simulink model "youBot_Arm_recovery"  (R2024a)
settings: Solver=ode15s  StartTime=0.0  StopTime=20  MaxStep=1e-2  RelTol=1e-3  AbsTol=1e-4
model workspace: external: MATLAB File youBot_DataFile.m (data not in the file)
undefined symbols (not defined in the file): Extr_Data_LinkHoles, Qt, s_curve_home2in, s_curve_in2out, s_curve_out2home, sigbuilder_block, smiData, X, Y, YBT_Par, Z
libraries: sm_lib x193, nesl_utility x130, fl_lib x53, simulink x13, Parts_Lib x10, MyMath_lib x8, Motor_Lib x5, Contact_Forces_Lib x4, ee_lib x2, sdl_lib x2
(part 5 of 8)

== system youBot_Arm_recovery/Arm/Environment/Load/Box ==
  Box : sm_lib/Body Elements/Brick Solid  BrickDimensions=[1 1 1]*YBT_Par.Cube.d  BrickDimensionsUnits=m  ExportEntireGeometry=off  InertiaType=CalculateFromGeometry  BasedOnType=Density  Density=1000  DensityUnits=kg/m^3  Mass=1  MassUnits=kg  CenterOfMass=[0 0 0]  CenterOfMassUnits=m  MomentsOfInertia=[1 1 1]  MomentsOfInertiaUnits=kg*m^2  ProductsOfInertia=[1 1 1]  ProductsOfInertiaUnits=kg*m^2  GraphicType=FromGeometry  MarkerShape=Sphere  MarkerSize=10  GraphicVisPropType=SimpleVisualProperties  GraphicDiffuseColor=[0.4 0.8 1.0]  GraphicOpacity=1.0  GraphicSpecularColor=[0.5 0.5 0.5 1.0]  GraphicAmbientColor=[0.15 0.15 0.15 1.0]  GraphicEmissiveColor=[0.0 0.0 0.0 1.0]  GraphicShininess=75  DoExposeReferenceFrame=on  SerializedFrames=<Frames/>
  Camera Frames : Subsystem
  Init Box 6-DOF Joint : sm_lib/Joints/6-DOF Joint  JointMode=Normal  CompositeWrenchDir=FollowerOnBase  CompositeWrenchFrame=BaseFrame  SenseConstraintForce=off  SenseConstraintTorque=off  SenseTotalForce=off  SenseTotalTorque=off  PxPositionTargetSpecify=off  PxPositionTargetPriority=High  PxPositionTargetValue=0  PxPositionTargetValueUnits=m  PxVelocityTargetSpecify=off  PxVelocityTargetPriority=High  PxVelocityTargetValue=0  PxVelocityTargetValueUnits=m/s  PxEquilibriumPosition=0  PxEquilibriumPositionUnits=m  PxSpringStiffness=0  PxSpringStiffnessUnits=N/m  PxDampingCoefficient=0  PxDampingCoefficientUnits=N/(m/s)  PxLowerLimitSpecify=off  PxLowerLimitBound=-1  PxLowerLimitBoundUnits=m  PxLowerLimitStiffness=1e6  PxLowerLimitStiffnessUnits=N/m  PxLowerLimitDamping=1e3  PxLowerLimitDampingUnits=N/(m/s)  PxLowerLimitTransitionRegionWidth=1e-4  PxLowerLimitTransitionRegionWidthUnits=m  PxUpperLimitSpecify=off  PxUpperLimitBound=1  PxUpperLimitBoundUnits=m  PxUpperLimitStiffness=1e6  PxUpperLimitStiffnessUnits=N/m  PxUpperLimitDamping=1e3  PxUpperLimitDampingUnits=N/(m/s)  PxUpperLimitTransitionRegionWidth=1e-4  PxUpperLimitTransitionRegionWidthUnits=m  PxTorqueActuationMode=NoTorque  PxMotionActuationMode=ComputedMotion  PxSensePosition=off  PxSenseVelocity=off  PxSenseAcceleration=off  PxSenseTorqueForce=off  PxSenseLowerLimitTorqueForce=off  PxSenseUpperLimitTorqueForce=off  PyPositionTargetSpecify=on  PyPositionTargetPriority=High  PyPositionTargetValue=YBT_Par.Cube.init_y  PyPositionTargetValueUnits=m  PyVelocityTargetSpecify=off  PyVelocityTargetPriority=High  PyVelocityTargetValue=0  PyVelocityTargetValueUnits=m/s  PyEquilibriumPosition=0  PyEquilibriumPositionUnits=m  PySpringStiffness=0  PySpringStiffnessUnits=N/m  PyDampingCoefficient=0  PyDampingCoefficientUnits=N/(m/s)  PyLowerLimitSpecify=off  PyLowerLimitBound=-1  PyLowerLimitBoundUnits=m  PyLowerLimitStiffness=1e6  PyLowerLimitStiffnessUnits=N/m  PyLowerLimitDamping=1e3  PyLowerLimitDampingUnits=N/(m/s)  PyLowerLimitTransitionRegionWidth=1e-4  PyLowerLimitTransitionRegionWidthUnits=m  PyUpperLimitSpecify=off  PyUpperLimitBound=1  PyUpperLimitBoundUnits=m  PyUpperLimitStiffness=1e6  PyUpperLimitStiffnessUnits=N/m  PyUpperLimitDamping=1e3  PyUpperLimitDampingUnits=N/(m/s)  PyUpperLimitTransitionRegionWidth=1e-4  PyUpperLimitTransitionRegionWidthUnits=m  PyTorqueActuationMode=NoTorque  PyMotionActuationMode=ComputedMotion  PySensePosition=off  PySenseVelocity=off  PySenseAcceleration=off  PySenseTorqueForce=off  PySenseLowerLimitTorqueForce=off  PySenseUpperLimitTorqueForce=off  PzPositionTargetSpecify=on  PzPositionTargetPriority=High  PzPositionTargetValue=(YBT_Par.Cube.d)/2+YBT_Par.Cube.init_z  PzPositionTargetValueUnits=m  PzVelocityTargetSpecify=off  PzVelocityTargetPriority=High  PzVelocityTargetValue=0  PzVelocityTargetValueUnits=m/s  PzEquilibriumPosition=0  PzEquilibriumPositionUnits=m  PzSpringStiffness=0  PzSpringStiffnessUnits=N/m  PzDampingCoefficient=0  PzDampingCoefficientUnits=N/(m/s)  PzLowerLimitSpecify=off  PzLowerLimitBound=-1  PzLowerLimitBoundUnits=m  PzLowerLimitStiffness=1e6  PzLowerLimitStiffnessUnits=N/m  PzLowerLimitDamping=1e3  PzLowerLimitDampingUnits=N/(m/s)  PzLowerLimitTransitionRegionWidth=1e-4  PzLowerLimitTransitionRegionWidthUnits=m  PzUpperLimitSpecify=off  PzUpperLimitBound=1  PzUpperLimitBoundUnits=m  PzUpperLimitStiffness=1e6  PzUpperLimitStiffnessUnits=N/m  PzUpperLimitDamping=1e3  PzUpperLimitDampingUnits=N/(m/s)  PzUpperLimitTransitionRegionWidth=1e-4  PzUpperLimitTransitionRegionWidthUnits=m  PzTorqueActuationMode=NoTorque  PzMotionActuationMode=ComputedMotion  PzSensePosition=off  PzSenseVelocity=off  PzSenseAcceleration=off  PzSenseTorqueForce=off  PzSenseLowerLimitTorqueForce=off  PzSenseUpperLimitTorqueForce=off  SphPositionTargetSpecify=on  SphPositionTargetPriority=High  SphPositionTargetRotationMethod=StandardAxis  SphPositionTargetFollAlignAxisA=+X  SphPositionTargetBaseAlignAxisA=+Y  SphPositionTargetFollAlignAxisB=+Y  SphPositionTargetBaseAlignAxisB=+Z  SphPositionTargetRotationStandardAxis=+X  SphPositionTargetRotationAngle=0  SphPositionTargetRotationAngleUnits=deg  SphPositionTargetRotationArbitraryAxis=[0 0 1]  SphPositionTargetRotationSequenceAxes=FollowerAxes  SphPositionTargetRotationSequence=XYX  SphPositionTargetRotationSequenceAngles=[0 0 0]  SphPositionTargetRotationSequenceAnglesUnits=deg  SphPositionTargetRotationMatrix=[1 0 0; 0 1 0; 0 0 1]  SphPositionTargetQuaternion=[1 0 0 0]  SphVelocityTargetSpecify=off  SphVelocityTargetPriority=High  SphVelocityTargetValue=[0 0 0]  SphVelocityTargetValueUnits=deg/s  SphVelocityTargetInFollowerFrame=on  SphEqPosRotationMethod=None  SphEqPosFollAlignAxisA=+X  SphEqPosBaseAlignAxisA=+Y  SphEqPosFollAlignAxisB=+Y  SphEqPosBaseAlignAxisB=+Z  SphEqPosRotationStandardAxis=+Z  SphEqPosRotationAngle=0.0  SphEqPosRotationAngleUnits=deg  SphEqPosRotationArbitraryAxis=[0 0 1]  SphEqPosRotationSequenceAxes=FollowerAxes  SphEqPosRotationSequence=XYX  SphEqPosRotationSequenceAngles=[0 0 0]  SphEqPosRotationSequenceAnglesUnits=deg  SphEqPosRotationMatrix=[1 0 0; 0 1 0; 0 0 1]  SphEqPosQuaternion=[1 0 0 0]  SphSpringStiffness=0  SphSpringStiffnessUnits=N*m/deg  SphDampingCoefficient=0  SphDampingCoefficientUnits=N*m/(deg/s)  SphLowerLimitSpecify=off  SphLowerLimitBound=15  SphLowerLimitBoundUnits=deg  SphLowerLimitStiffness=1e4  SphLowerLimitStiffnessUnits=N*m/deg  SphLowerLimitDamping=10  SphLowerLimitDampingUnits=N*m/(deg/s)  SphLowerLimitTransitionRegionWidth=0.1  SphLowerLimitTransitionRegionWidthUnits=deg  SphUpperLimitSpecify=off  SphUpperLimitBound=45  SphUpperLimitBoundUnits=deg  SphUpperLimitStiffness=1e4  SphUpperLimitStiffnessUnits=N*m/deg  SphUpperLimitDamping=10  SphUpperLimitDampingUnits=N*m/(deg/s)  SphUpperLimitTransitionRegionWidth=0.1  SphUpperLimitTransitionRegionWidthUnits=deg  SphTorqueActuationMode=NoTorque  SphActuateTorqueX=off  SphActuateTorqueY=off  SphActuateTorqueZ=off  SphActuateTorque=off  SphActuationFrame=BaseFrame  SphSensePosition=off  SphSenseVelocityX=off  SphSenseVelocityY=off  SphSenseVelocityZ=off  SphSenseVelocity=off  SphSenseAccelerationX=off  SphSenseAccelerationY=off  SphSenseAccelerationZ=off  SphSenseAcceleration=off  SphSenseLowerLimitTorqueMag=off  SphSenseUpperLimitTorqueMag=off  SphSensingFrame=BaseFrame
  Marks : Subsystem
  Transform Face nx : sm_lib/Frames and Transforms/Rigid Transform  RotationMethod=StandardAxis  FollAlignAxisA=+X  BaseAlignAxisA=+Y  FollAlignAxisB=+Y  BaseAlignAxisB=+Z  RotationStandardAxis=+Y  RotationAngle=-90  RotationAngleUnits=deg  RotationArbitraryAxis=[0 0 1]  RotationSequenceAxes=FollowerAxes  RotationSequence=XYX  RotationSequenceAngles=[0 0 0]  RotationSequenceAnglesUnits=deg  RotationMatrix=[1 0 0; 0 1 0; 0 0 1]  Quaternion=[1 0 0 0]  TranslationMethod=None  TranslationCartesianOffset=[0 0 0]  TranslationCartesianOffsetUnits=m  TranslationStandardAxis=+Z  TranslationStandardOffset=0  TranslationStandardOffsetUnits=m  TranslationROffset=0  TranslationROffsetUnits=m  TranslationThetaOffset=0  TranslationThetaOffsetUnits=deg  TranslationZOffset=0  TranslationZOffsetUnits=m
  Transform Face px : sm_lib/Frames and Transforms/Rigid Transform  RotationMethod=StandardAxis  FollAlignAxisA=+X  BaseAlignAxisA=+Y  FollAlignAxisB=+Y  BaseAlignAxisB=+Z  RotationStandardAxis=+Y  RotationAngle=90  RotationAngleUnits=deg  RotationArbitraryAxis=[0 0 1]  RotationSequenceAxes=FollowerAxes  RotationSequence=XYX  RotationSequenceAngles=[0 0 0]  RotationSequenceAnglesUnits=deg  RotationMatrix=[1 0 0; 0 1 0; 0 0 1]  Quaternion=[1 0 0 0]  TranslationMethod=None  TranslationCartesianOffset=[0 0 0]  TranslationCartesianOffsetUnits=m  TranslationStandardAxis=+Z  TranslationStandardOffset=0  TranslationStandardOffsetUnits=m  TranslationROffset=0  TranslationROffsetUnits=m  TranslationThetaOffset=0  TranslationThetaOffsetUnits=deg  TranslationZOffset=0  TranslationZOffsetUnits=m
  Fa : PMIOPort  Side=Right
  Ctr : PMIOPort  Port=2  Side=Left
  Fb : PMIOPort  Port=3  Side=Right
  W : PMIOPort  Port=4  Side=Left
  connections:
  Init Box 6-DOF Joint/LConn1 -- W/RConn1
  Box/RConn1 -- Transform Face px/LConn1 -- Transform Face nx/LConn1 -- Ctr/RConn1 -- Init Box 6-DOF Joint/RConn1 -- Marks/LConn1 -- Camera Frames/LConn1
  Fb/RConn1 -- Transform Face nx/RConn1
  Fa/RConn1 -- Transform Face px/RConn1

== system youBot_Arm_recovery/Arm/Environment/Load/None ==
  Invisible Mass : sm_lib/Body Elements/Brick Solid  BrickDimensions=[1 1 1]  BrickDimensionsUnits=cm  ExportEntireGeometry=off  InertiaType=CalculateFromGeometry  BasedOnType=Density  Density=1000  DensityUnits=kg/m^3  Mass=1  MassUnits=kg  CenterOfMass=[0 0 0]  CenterOfMassUnits=m  MomentsOfInertia=[1 1 1]  MomentsOfInertiaUnits=kg*m^2  ProductsOfInertia=[1 1 1]  ProductsOfInertiaUnits=kg*m^2  GraphicType=FromGeometry  MarkerShape=Sphere  MarkerSize=10  GraphicVisPropType=SimpleVisualProperties  GraphicDiffuseColor=[0.5 0.5 0.5]  GraphicOpacity=0  GraphicSpecularColor=[0.5 0.5 0.5 1.0]  GraphicAmbientColor=[0.15 0.15 0.15 1.0]  GraphicEmissiveColor=[0.0 0.0 0.0 1.0]  GraphicShininess=75  DoExposeReferenceFrame=on  SerializedFrames=<Frames/>
  Transform Box : sm_lib/Frames and Transforms/Rigid Transform  RotationMethod=None  FollAlignAxisA=+X  BaseAlignAxisA=+Y  FollAlignAxisB=+Y  BaseAlignAxisB=+Z  RotationStandardAxis=+Z  RotationAngle=0.0  RotationAngleUnits=deg  RotationArbitraryAxis=[0 0 1]  RotationSequenceAxes=FollowerAxes  RotationSequence=XYX  RotationSequenceAngles=[0 0 0]  RotationSequenceAnglesUnits=deg  RotationMatrix=[1 0 0; 0 1 0; 0 0 1]  Quaternion=[1 0 0 0]  TranslationMethod=Cartesian  TranslationCartesianOffset=[0 YBT_Par.Cube.init_y YBT_Par.Cube.init_z+YBT_Par.Cube.d/2]  TranslationCartesianOffsetUnits=m  TranslationStandardAxis=+Z  TranslationStandardOffset=0  TranslationStandardOffsetUnits=m  TranslationROffset=0  TranslationROffsetUnits=m  TranslationThetaOffset=0  TranslationThetaOffsetUnits=deg  TranslationZOffset=0  TranslationZOffsetUnits=m
  Fa : PMIOPort  Side=Right
  Ctr : PMIOPort  Port=2  Side=Left
  Fb : PMIOPort  Port=3  Side=Right
  W : PMIOPort  Port=4  Side=Left
  connections:
  Transform Box/RConn1 -- Invisible Mass/RConn1 -- Ctr/RConn1
  Transform Box/LConn1 -- W/RConn1

== system youBot_Arm_recovery/Input/Control/Joint Commands/BeltIn to BeltOut ==
  t : Inport
  Bicep : Lookup_n-D  NumberOfTableDimensions=1  LookupTableObject=''  BreakpointsForDimension1=s_curve_in2out.t  Table=s_curve_in2out.q(2,:)  InterpMethod=Cubic spline  ExtrapMethod=Clip  InternalRulePriority=Speed  RndMeth=Simplest
  Forearm : Lookup_n-D  NumberOfTableDimensions=1  LookupTableObject=''  BreakpointsForDimension1=s_curve_in2out.t  Table=s_curve_in2out.q(3,:)  InterpMethod=Cubic spline  ExtrapMethod=Clip  InternalRulePriority=Speed  RndMeth=Simplest
  Gripper : Lookup_n-D  NumberOfTableDimensions=1  LookupTableObject=''  BreakpointsForDimension1=in2out.t  Table=in2out.q(5,:)  InterpMethod=Cubic spline  ExtrapMethod=Clip  InternalRulePriority=Speed  RndMeth=Simplest
  Mux : Mux  Inputs=5
  Pivot : Lookup_n-D  NumberOfTableDimensions=1  LookupTableObject=''  BreakpointsForDimension1=s_curve_in2out.t  Table=s_curve_in2out.q(1,:)  InterpMethod=Cubic spline  ExtrapMethod=Clip  InternalRulePriority=Speed  RndMeth=Simplest
  Wrist : Lookup_n-D  NumberOfTableDimensions=1  LookupTableObject=''  BreakpointsForDimension1=s_curve_in2out.t  Table=s_curve_in2out.q(4,:)  InterpMethod=Cubic spline  ExtrapMethod=Clip  InternalRulePriority=Speed  RndMeth=Simplest
  q : Outport  VectorParamsAs1DForOutWhenUnconnected=off
  wires:
  Pivot/1 -> Mux/1
  t/1 -> Gripper/1, Wrist/1, Forearm/1, Bicep/1, Pivot/1
  Bicep/1 -> Mux/2
  Mux/1 -> q/1
  Forearm/1 -> Mux/3
  Wrist/1 -> Mux/4
  Gripper/1 -> Mux/5

== system youBot_Arm_recovery/Input/Control/Joint Commands/BeltOut to Home ==
  t : Inport
  Bicep : Lookup_n-D  NumberOfTableDimensions=1  LookupTableObject=''  BreakpointsForDimension1=s_curve_out2home.t  Table=s_curve_out2home.q(2,:)  InterpMethod=Cubic spline  ExtrapMethod=Clip  InternalRulePriority=Speed  RndMeth=Simplest
  Forearm : Lookup_n-D  NumberOfTableDimensions=1  LookupTableObject=''  BreakpointsForDimension1=s_curve_out2home.t  Table=s_curve_out2home.q(3,:)  InterpMethod=Cubic spline  ExtrapMethod=Clip  InternalRulePriority=Speed  RndMeth=Simplest
  Gripper : Lookup_n-D  NumberOfTableDimensions=1  LookupTableObject=''  BreakpointsForDimension1=out2home.t  Table=out2home.q(5,:)  InterpMethod=Cubic spline  ExtrapMethod=Clip  InternalRulePriority=Speed  RndMeth=Simplest
  Mux : Mux  Inputs=5
  Pivot : Lookup_n-D  NumberOfTableDimensions=1  LookupTableObject=''  BreakpointsForDimension1=s_curve_out2home.t  Table=s_curve_out2home.q(1,:)  InterpMethod=Cubic spline  ExtrapMethod=Clip  InternalRulePriority=Speed  RndMeth=Simplest
  Wrist : Lookup_n-D  NumberOfTableDimensions=1  LookupTableObject=''  BreakpointsForDimension1=s_curve_out2home.t  Table=s_curve_out2home.q(4,:)  InterpMethod=Cubic spline  ExtrapMethod=Clip  InternalRulePriority=Speed  RndMeth=Simplest
  q : Outport  VectorParamsAs1DForOutWhenUnconnected=off
  wires:
  Gripper/1 -> Mux/5
  Wrist/1 -> Mux/4
  Forearm/1 -> Mux/3
  Mux/1 -> q/1
  Bicep/1 -> Mux/2
  t/1 -> Pivot/1, Bicep/1, Forearm/1, Wrist/1, Gripper/1
  Pivot/1 -> Mux/1

== system youBot_Arm_recovery/Input/Control/Joint Commands/Home to BeltIn ==
  t : Inport
  Bicep : Lookup_n-D  NumberOfTableDimensions=1  LookupTableObject=''  BreakpointsForDimension1=s_curve_home2in.t  Table=s_curve_home2in.q(2,:)  InterpMethod=Cubic spline  ExtrapMethod=Clip  InternalRulePriority=Speed  RndMeth=Simplest
  Forearm : Lookup_n-D  NumberOfTableDimensions=1  LookupTableObject=''  BreakpointsForDimension1=s_curve_home2in.t  Table=s_curve_home2in.q(3,:)  InterpMethod=Cubic spline  ExtrapMethod=Clip  InternalRulePriority=Speed  RndMeth=Simplest
  Gripper : Lookup_n-D  NumberOfTableDimensions=1  LookupTableObject=''  BreakpointsForDimension1=home2in.t  Table=home2in.q(5,:)  InterpMethod=Cubic spline  ExtrapMethod=Clip  InternalRulePriority=Speed  RndMeth=Simplest
  Mux : Mux  Inputs=5
  Pivot : Lookup_n-D  NumberOfTableDimensions=1  LookupTableObject=''  BreakpointsForDimension1=s_curve_home2in.t  Table=s_curve_home2in.q(1,:)  InterpMethod=Cubic spline  ExtrapMethod=Clip  InternalRulePriority=Speed  RndMeth=Simplest
  Wrist : Lookup_n-D  NumberOfTableDimensions=1  LookupTableObject=''  BreakpointsForDimension1=s_curve_home2in.t  Table=s_curve_home2in.q(4,:)  InterpMethod=Cubic spline  ExtrapMethod=Clip  InternalRulePriority=Speed  RndMeth=Simplest
  q : Outport  VectorParamsAs1DForOutWhenUnconnected=off
  wires:
  Gripper/1 -> Mux/5
  Wrist/1 -> Mux/4
  Forearm/1 -> Mux/3
  Mux/1 -> q/1
  Bicep/1 -> Mux/2
  t/1 -> Pivot/1, Bicep/1, Forearm/1, Wrist/1, Gripper/1
  Pivot/1 -> Mux/1

== system youBot_Arm_recovery/Input/Control Belt/Robot Commands/Subsystem ==
  In1 : Inport
  Demux : Demux  Tag=STV Demux  Outputs=7
      settings: DisplayOption=none
  cP : Outport  Tag=STV Outport  VectorParamsAs1DForOutWhenUnconnected=off
  cB : Outport  Tag=STV Outport  Port=2  VectorParamsAs1DForOutWhenUnconnected=off
  cF : Outport  Tag=STV Outport  Port=3  VectorParamsAs1DForOutWhenUnconnected=off
  cW : Outport  Tag=STV Outport  Port=4  VectorParamsAs1DForOutWhenUnconnected=off
  cG : Outport  Tag=STV Outport  Port=5  VectorParamsAs1DForOutWhenUnconnected=off
  ca : Outport  Tag=STV Outport  Port=6  VectorParamsAs1DForOutWhenUnconnected=off
  cb : Outport  Tag=STV Outport  Port=7  VectorParamsAs1DForOutWhenUnconnected=off
  wires:
  Demux/7 -> cb/1
  Demux/6 -> ca/1
  Demux/5 -> cG/1
  Demux/4 -> cW/1
  Demux/3 -> cF/1
  Demux/2 -> cB/1
  Demux/1 -> cP/1
  In1/1 -> Demux/1

== system youBot_Arm_recovery/Input/Signals/Belt Commands/Subsystem ==
  In1 : Inport
  Demux : Demux  Tag=STV Demux  Outputs=2
      settings: DisplayOption=none
  Belt In On : Outport  Tag=STV Outport  VectorParamsAs1DForOutWhenUnconnected=off
  Belt Out On : Outport  Tag=STV Outport  Port=2  VectorParamsAs1DForOutWhenUnconnected=off
  wires:
  Demux/1 -> Belt In On/1
  Demux/2 -> Belt Out On/1
  In1/1 -> Demux/1

== system youBot_Arm_recovery/Input/Signals/Robot Commands/Subsystem ==
  In1 : Inport
  Demux : Demux  Tag=STV Demux  Outputs=7
      settings: DisplayOption=none
  cP : Outport  Tag=STV Outport  VectorParamsAs1DForOutWhenUnconnected=off
  cB : Outport  Tag=STV Outport  Port=2  VectorParamsAs1DForOutWhenUnconnected=off
  cF : Outport  Tag=STV Outport  Port=3  VectorParamsAs1DForOutWhenUnconnected=off
  cW : Outport  Tag=STV Outport  Port=4  VectorParamsAs1DForOutWhenUnconnected=off
  cG : Outport  Tag=STV Outport  Port=5  VectorParamsAs1DForOutWhenUnconnected=off
  ca : Outport  Tag=STV Outport  Port=6  VectorParamsAs1DForOutWhenUnconnected=off
  cb : Outport  Tag=STV Outport  Port=7  VectorParamsAs1DForOutWhenUnconnected=off
  wires:
  In1/1 -> Demux/1
  Demux/1 -> cP/1
  Demux/2 -> cB/1
  Demux/3 -> cF/1
  Demux/4 -> cW/1
  Demux/5 -> cG/1
  Demux/6 -> ca/1
  Demux/7 -> cb/1

== system youBot_Arm_recovery/Arm/Actuation/Motor/Bicep/Ideal ==
  C : Inport
  Current Source : fl_lib/Electrical/Electrical Sources/Controlled Current Source
  Meas B : Subsystem
      mask Display: disp('m')
  PS Abs : MyMath_lib/PS Abs
      settings: InternalSimscapePortConfiguration="{\"Bottom\":[],\"Left\":[{\"id\":\"I\",\"label\":\"\",\"type\":\"input\"}],\"Right\":[{\"id\":\"O\",\"label\":\"\",\"type\":\"output\"}],\"Top\":[]}"
  PS Motor Const : fl_lib/Physical Signals/Functions/PS Gain  gain=YBT_Par.Bicep.Motor.K/YBT_Par.Bicep.Motor.gr s^2 / (kg*m^2)
  Resistor : fl_lib/Electrical/Electrical Elements/Resistor  R=YBT_Par.Bicep.Motor.R Ohm  i_specify=off  i_priority=None  i=0 A  i_nominal_specify=off  i_nominal_value=1  i_nominal_unit=A  v_specify=off  v_priority=None  v=0 V  v_nominal_specify=off  v_nominal_value=1  v_nominal_unit=V
  RevolutePivotBicep : sm_lib/Joints/Revolute Joint  JointMode=Normal  CompositeWrenchDir=FollowerOnBase  CompositeWrenchFrame=BaseFrame  SenseConstraintForce=on  SenseConstraintTorque=off  SenseTotalForce=off  SenseTotalTorque=off  PositionTargetSpecify=on  PositionTargetPriority=Low  PositionTargetValue=smiData.RevoluteJoint(1).Rz.Pos  PositionTargetValueUnits=deg  VelocityTargetSpecify=off  VelocityTargetPriority=High  VelocityTargetValue=0  VelocityTargetValueUnits=deg/s  EquilibriumPosition=0  EquilibriumPositionUnits=rad  SpringStiffness=0  SpringStiffnessUnits=N*m/rad  DampingCoefficient=YBT_Par.Bicep.Motor.friction  DampingCoefficientUnits=N*m/(rad/s)  LowerLimitSpecify=off  LowerLimitBound=-90  LowerLimitBoundUnits=deg  LowerLimitStiffness=1e4  LowerLimitStiffnessUnits=N*m/deg  LowerLimitDamping=10  LowerLimitDampingUnits=N*m/(deg/s)  LowerLimitTransitionRegionWidth=0.1  LowerLimitTransitionRegionWidthUnits=deg  UpperLimitSpecify=off  UpperLimitBound=90  UpperLimitBoundUnits=deg  UpperLimitStiffness=1e4  UpperLimitStiffnessUnits=N*m/deg  UpperLimitDamping=10  UpperLimitDampingUnits=N*m/(deg/s)  UpperLimitTransitionRegionWidth=0.1  UpperLimitTransitionRegionWidthUnits=deg  TorqueActuationMode=ComputedTorque  MotionActuationMode=InputMotion  SensePosition=on  SenseVelocity=on  SenseAcceleration=off  SenseTorqueForce=on  SenseLowerLimitTorqueForce=off  SenseUpperLimitTorqueForce=off
  Simulink-PS Converter4 : nesl_utility/Simulink-PS Converter  Tag=CustomStyle  PhysicalDomain=network_engine_domain  SubClassName=ps_input  LeftPortType=input  RightPortType=output  PseudoPeriodic=off  Frequencies=[]  NoiseDistribution=none  NoiseParameters=[]  Unit=deg  AffineConversion=off  FilteringAndDerivatives=filter  SimscapeFilterOrder=2  InputFilterTimeConstant=0.005  UdotUserProvided=1
  B : PMIOPort  Side=Left
  F : PMIOPort  Port=2  Side=Right
  + : PMIOPort  Port=3  Side=Left
  - : PMIOPort  Port=4  Side=Right
  m : Outport  VectorParamsAs1DForOutWhenUnconnected=off
  wires:
  Meas B/1(B) -> m/1
  C/1 -> Simulink-PS Converter4/1
  connections:
  RevolutePivotBicep/RConn3 -- Meas B/LConn2
  RevolutePivotBicep/RConn4 -- PS Motor Const/LConn1 -- Meas B/LConn3
  RevolutePivotBicep/RConn2 -- Meas B/LConn1
  PS Abs/RConn1 -- Meas B/LConn5 -- Current Source/RConn1
  +/RConn1 -- Current Source/RConn2
  Resistor/LConn1 -- Current Source/LConn1
  PS Motor Const/RConn1 -- PS Abs/LConn1
  -/RConn1 -- Resistor/RConn1
  RevolutePivotBicep/LConn1 -- B/RConn1
  RevolutePivotBicep/RConn1 -- F/RConn1
  RevolutePivotBicep/LConn2 -- Simulink-PS Converter4/RConn1
  RevolutePivotBicep/RConn5 -- Meas B/LConn4

== system youBot_Arm_recovery/Arm/Actuation/Motor/Bicep/Motor ==
  C : Inport
  Meas P : Subsystem  Tag=CustomStyle
      mask Display: disp('m')
  Motor : Motor_Lib/Motor  VariantControl=Motor  r_motor=YBT_Par.Bicep.Motor.R  l_motor=YBT_Par.Bicep.Motor.L  k_motor=1/YBT_Par.Bicep.Motor.K  i_motor_noLoad=YBT_Par.Bicep.Motor.no_load_i  v_supply=YBT_Par.Battery.v  gear_ratio=YBT_Par.Bicep.Motor.gr  friction_visc=YBT_Par.Bicep.Motor.friction  ctrl_deadZone=YBT_Par.Control.Dead_Band
  RevolutePivotBicep : sm_lib/Joints/Revolute Joint  JointMode=Normal  CompositeWrenchDir=FollowerOnBase  CompositeWrenchFrame=BaseFrame  SenseConstraintForce=on  SenseConstraintTorque=off  SenseTotalForce=off  SenseTotalTorque=off  PositionTargetSpecify=on  PositionTargetPriority=Low  PositionTargetValue=smiData.RevoluteJoint(1).Rz.Pos  PositionTargetValueUnits=deg  VelocityTargetSpecify=off  VelocityTargetPriority=High  VelocityTargetValue=0  VelocityTargetValueUnits=deg/s  EquilibriumPosition=0  EquilibriumPositionUnits=rad  SpringStiffness=0  SpringStiffnessUnits=N*m/rad  DampingCoefficient=YBT_Par.Bicep.Motor.friction*0  DampingCoefficientUnits=N*m/(rad/s)  LowerLimitSpecify=off  LowerLimitBound=-90  LowerLimitBoundUnits=deg  LowerLimitStiffness=1e4  LowerLimitStiffnessUnits=N*m/deg  LowerLimitDamping=10  LowerLimitDampingUnits=N*m/(deg/s)  LowerLimitTransitionRegionWidth=0.1  LowerLimitTransitionRegionWidthUnits=deg  UpperLimitSpecify=off  UpperLimitBound=90  UpperLimitBoundUnits=deg  UpperLimitStiffness=1e4  UpperLimitStiffnessUnits=N*m/deg  UpperLimitDamping=10  UpperLimitDampingUnits=N*m/(deg/s)  UpperLimitTransitionRegionWidth=0.1  UpperLimitTransitionRegionWidthUnits=deg  TorqueActuationMode=InputTorque  MotionActuationMode=ComputedMotion  SensePosition=on  SenseVelocity=on  SenseAcceleration=off  SenseTorqueForce=on  SenseLowerLimitTorqueForce=off  SenseUpperLimitTorqueForce=off
  Sensing i : Subsystem
      mask Display: disp('i')
  B : PMIOPort  Side=Left
  F : PMIOPort  Port=2  Side=Right
  - : PMIOPort  Port=3  Side=Right
  + : PMIOPort  Port=4  Side=Left
  m : Outport  VectorParamsAs1DForOutWhenUnconnected=off
  wires:
  Meas P/1(m) -> m/1
  C/1 -> Motor/1
  connections:
  RevolutePivotBicep/RConn2 -- Motor/RConn1 -- Meas P/LConn1
  Meas P/LConn3 -- RevolutePivotBicep/RConn4
  RevolutePivotBicep/RConn3 -- Motor/RConn2 -- Meas P/LConn2
  Motor/LConn1 -- RevolutePivotBicep/LConn2
  RevolutePivotBicep/RConn1 -- F/RConn1
  RevolutePivotBicep/LConn1 -- B/RConn1
  Motor/RConn3 -- Sensing i/LConn1
  Motor/LConn2 -- +/RConn1
  -/RConn1 -- Sensing i/RConn2
  Meas P/LConn5 -- Sensing i/RConn1
  RevolutePivotBicep/RConn5 -- Meas P/LConn4

== system youBot_Arm_recovery/Arm/Actuation/Motor/Bicep/Test Motor ==
  C : Inport
  Current Source : fl_lib/Electrical/Electrical Sources/Controlled Current Source
  DC Motor : ee_lib/Electromechanical/Brushed Motors/DC Motor  field_option=ee.enum.field_option.pm  Rf=100 Ohm  Lf=1 H  Laf=0.15 H  If0=0 A  parameterization=1  Ra=YBT_Par.Bicep.Motor.R Ohm  La=YBT_Par.Bicep.Motor.L H  emf_or_torque=2  Kv=YBT_Par.Pivot.Motor.K V/rpm  Ki=1/YBT_Par.Bicep.Motor.K N*m/A  T_stall=2.4e-4 N*m  w_max=1.91e+4 rpm  w_rated=1.5e+4 rpm  P_rated=0.08 W  V_rated=1.5 V  lam_param=2  i_noload=YBT_Par.Bicep.Motor.no_load_i A  V_i_noload=24 V  J=0 g*cm^2  lam=0 N*m/(rad/s)  speed0=0 rpm  enable_fault_armature=simscape.enum.onoff.off  rev_faulted=1 / 3  G_faulted_armature=1e-5 S  fault_trigger_armature=ee.enum.faults.faultTrigger.temporal  t_fault_armature=1 s  max_permissible_current_armature=inf A  t_fail_on_current_armature=1 s  enable_fault_field=simscape.enum.onoff.off  G_faulted_field=1e-5 S  fault_trigger_field=ee.enum.faults.faultTrigger.temporal  t_fault_field=1 s  max_permissible_current_field=inf A  t_fail_on_current_field=1 s  fault_action=simscape.enum.assert.action.none  alpha=3.93e-3 1/K  Tmeas=25 degC  thermal_mass=100 J/K  initial_temperature=25 degC
  MRRef : fl_lib/Mechanical/Rotational Elements/Mechanical Rotational Reference
  Meas P : Subsystem  Tag=CustomStyle
      mask Display: disp('m')
  PS Motor Const : fl_lib/Physical Signals/Functions/PS Gain  gain=YBT_Par.Bicep.Motor.K/YBT_Par.Bicep.Motor.gr s^2 / (kg*m^2)
  RevolutePivotBicep : sm_lib/Joints/Revolute Joint  JointMode=Normal  CompositeWrenchDir=FollowerOnBase  CompositeWrenchFrame=BaseFrame  SenseConstraintForce=on  SenseConstraintTorque=off  SenseTotalForce=off  SenseTotalTorque=off  PositionTargetSpecify=on  PositionTargetPriority=Low  PositionTargetValue=smiData.RevoluteJoint(1).Rz.Pos  PositionTargetValueUnits=deg  VelocityTargetSpecify=off  VelocityTargetPriority=High  VelocityTargetValue=0  VelocityTargetValueUnits=deg/s  EquilibriumPosition=0  EquilibriumPositionUnits=rad  SpringStiffness=0  SpringStiffnessUnits=N*m/rad  DampingCoefficient=YBT_Par.Bicep.Motor.friction  DampingCoefficientUnits=N*m/(rad/s)  LowerLimitSpecify=off  LowerLimitBound=-90  LowerLimitBoundUnits=deg  LowerLimitStiffness=1e4  LowerLimitStiffnessUnits=N*m/deg  LowerLimitDamping=10  LowerLimitDampingUnits=N*m/(deg/s)  LowerLimitTransitionRegionWidth=0.1  LowerLimitTransitionRegionWidthUnits=deg  UpperLimitSpecify=off  UpperLimitBound=90  UpperLimitBoundUnits=deg  UpperLimitStiffness=1e4  UpperLimitStiffnessUnits=N*m/deg  UpperLimitDamping=10  UpperLimitDampingUnits=N*m/(deg/s)  UpperLimitTransitionRegionWidth=0.1  UpperLimitTransitionRegionWidthUnits=deg  TorqueActuationMode=ComputedTorque  MotionActuationMode=InputMotion  SensePosition=on  SenseVelocity=on  SenseAcceleration=off  SenseTorqueForce=on  SenseLowerLimitTorqueForce=off  SenseUpperLimitTorqueForce=off
  Rotational Damper : fl_lib/Mechanical/Rotational Elements/Rotational Damper  D=YBT_Par.Bicep.Motor.friction N*m/(rad/s)  w_specify=off  w_priority=None  w=0 rad/s  w_nominal_specify=off  w_nominal_value=1  w_nominal_unit=rad/s  t_specify=off  t_priority=None  t=0 N*m  t_nominal_specify=off  t_nominal_value=1  t_nominal_unit=N*m
  Simple Gear : sdl_lib/Gears/Simple Gear  ratio=YBT_Par.Bicep.Motor.gr  rotation_direction=3-2*(1)  enable_faults=simscape.enum.onoff.off  efficiency_fault=0.05  fault_angles=pi / 12 rad  friction_model=1  T_noload=0.1 N*m  T_nom=5 N*m  efficiency_nom=0.8  efficiency=0.8  temperature_TLU=[ 280 300 320 ] K  load_TLU=[ 1 5 10 ] N*m  efficiency_TLU=[ 0.95 0.9 0.85 ]  efficiency_TLU2=[ 0.85 0.8 0.75; 0.95 0.9 0.85; 0.85 0.8 0.7 ]  w_thr=0.01 rad/s  pwr_thr=0.001 W  enable_backlash=false  hardstop_model=simscape.enum.hardstop.smooth  backlash_distance=1e-3 mm  r_base=0.1 m  transition=1e-4 mm  backlash_stiffness=1e7 N/m  backlash_damping=1e6 N*s/m  coeff_rest=0  v_tol=0.001 m/s  f_tol=0 N  mu_visc=[ 0 0 ] N*m/(rad/s)  thermal_mass=50 J/K  temperature_specify=off  temperature_priority=High  temperature=300 K  temperature_nominal_specify=off  temperature_nominal_value=1  temperature_nominal_unit=K  x_backlash_specify=off  x_backlash_priority=None  x_backlash=0 mm  x_backlash_nominal_specify=off  x_backlash_nominal_value=1  x_backlash_nominal_unit=mm  f_hardstop_specify=off  f_hardstop_priority=None  f_hardstop=0 N  f_hardstop_nominal_specify=off  f_hardstop_nominal_value=1  f_hardstop_nominal_unit=N  v_backlash_specify=off  v_backlash_priority=None  v_backlash=0 m/s  v_backlash_nominal_specify=off  v_backlash_nominal_value=1  v_backlash_nominal_unit=m/s
  Simulink-PS Converter : nesl_utility/Simulink-PS Converter  Tag=CustomStyle  PhysicalDomain=network_engine_domain  SubClassName=ps_input  LeftPortType=input  RightPortType=output  PseudoPeriodic=off  Frequencies=[]  NoiseDistribution=none  NoiseParameters=[]  Unit=deg  AffineConversion=off  FilteringAndDerivatives=filter  SimscapeFilterOrder=2  InputFilterTimeConstant=0.005  UdotUserProvided=1
  B : PMIOPort  Side=Left
  F : PMIOPort  Port=2  Side=Right
  + : PMIOPort  Port=3  Side=Left
  - : PMIOPort  Port=4  Side=Right
  m : Outport  VectorParamsAs1DForOutWhenUnconnected=off
  wires:
  C/1 -> Simulink-PS Converter/1
  Meas P/1(P) -> m/1
  connections:
  RevolutePivotBicep/LConn1 -- B/RConn1
  RevolutePivotBicep/RConn1 -- F/RConn1
  RevolutePivotBicep/LConn2 -- Simulink-PS Converter/RConn1
  Current Source/RConn1 -- PS Motor Const/RConn1 -- Meas P/LConn5
  +/RConn1 -- Current Source/RConn2
  Current Source/LConn1 -- DC Motor/LConn1
  RevolutePivotBicep/RConn3 -- Meas P/LConn2
  RevolutePivotBicep/RConn4 -- PS Motor Const/LConn1 -- Meas P/LConn3
  RevolutePivotBicep/RConn2 -- Meas P/LConn1
  DC Motor/RConn1 -- -/RConn1
  DC Motor/RConn2 -- MRRef/LConn1 -- Rotational Damper/RConn1
  Simple Gear/LConn1 -- DC Motor/LConn2
  Rotational Damper/LConn1 -- Simple Gear/RConn1
  Meas P/LConn4 -- RevolutePivotBicep/RConn5

== system youBot_Arm_recovery/Arm/Actuation/Motor/Finger A/Meas a ==
  Bus Creator : BusCreator  Inputs=5
  PS-Simulink Converter : nesl_utility/PS-Simulink Converter  PhysicalDomain=network_engine_domain  SubClassName=ps_output  LeftPortType=input  RightPortType=output  PseudoPeriodic=off  Frequencies=[]  VectorFormat=1-D array  Unit=mm  AffineConversion=off
  PS-Simulink Converter1 : nesl_utility/PS-Simulink Converter  PhysicalDomain=network_engine_domain  SubClassName=ps_output  LeftPortType=input  RightPortType=output  PseudoPeriodic=off  Frequencies=[]  VectorFormat=1-D array  Unit=A  AffineConversion=off
  PS-Simulink Converter2 : nesl_utility/PS-Simulink Converter  PhysicalDomain=network_engine_domain  SubClassName=ps_output  LeftPortType=input  RightPortType=output  PseudoPeriodic=off  Frequencies=[]  VectorFormat=1-D array  Unit=1  AffineConversion=off
  PS-Simulink Converter7 : nesl_utility/PS-Simulink Converter  PhysicalDomain=network_engine_domain  SubClassName=ps_output  LeftPortType=input  RightPortType=output  PseudoPeriodic=off  Frequencies=[]  VectorFormat=1-D array  Unit=mm/s  AffineConversion=off
  PS-Simulink Converter8 : nesl_utility/PS-Simulink Converter  PhysicalDomain=network_engine_domain  SubClassName=ps_output  LeftPortType=input  RightPortType=output  PseudoPeriodic=off  Frequencies=[]  VectorFormat=1-D array  Unit=N  AffineConversion=off
  p : PMIOPort  Side=Left
  v : PMIOPort  Port=2  Side=Left
  f : PMIOPort  Port=3  Side=Left
  fc : PMIOPort  Port=4  Side=Left
  i : PMIOPort  Port=5  Side=Left
  m : Outport  VectorParamsAs1DForOutWhenUnconnected=off
  wires:
  PS-Simulink Converter/1 -> Bus Creator/1  "p"
  PS-Simulink Converter7/1 -> Bus Creator/2  "v"
  PS-Simulink Converter8/1 -> Bus Creator/3  "f"
  Bus Creator/1 -> m/1  "a"
  PS-Simulink Converter1/1 -> Bus Creator/4  "i"
  PS-Simulink Converter2/1 -> Bus Creator/5  "fc"
  connections:
  PS-Simulink Converter/LConn1 -- p/RConn1
  PS-Simulink Converter7/LConn1 -- v/RConn1
  PS-Simulink Converter8/LConn1 -- f/RConn1
  PS-Simulink Converter1/LConn1 -- i/RConn1
  PS-Simulink Converter2/LConn1 -- fc/RConn1

== system youBot_Arm_recovery/Arm/Actuation/Motor/Finger B/Meas b ==
  Bus Creator : BusCreator  Inputs=5
  PS-Simulink Converter : nesl_utility/PS-Simulink Converter  PhysicalDomain=network_engine_domain  SubClassName=ps_output  LeftPortType=input  RightPortType=output  PseudoPeriodic=off  Frequencies=[]  VectorFormat=1-D array  Unit=mm  AffineConversion=off
  PS-Simulink Converter1 : nesl_utility/PS-Simulink Converter  PhysicalDomain=network_engine_domain  SubClassName=ps_output  LeftPortType=input  RightPortType=output  PseudoPeriodic=off  Frequencies=[]  VectorFormat=1-D array  Unit=A  AffineConversion=off
  PS-Simulink Converter2 : nesl_utility/PS-Simulink Converter  PhysicalDomain=network_engine_domain  SubClassName=ps_output  LeftPortType=input  RightPortType=output  PseudoPeriodic=off  Frequencies=[]  VectorFormat=1-D array  Unit=1  AffineConversion=off
  PS-Simulink Converter7 : nesl_utility/PS-Simulink Converter  PhysicalDomain=network_engine_domain  SubClassName=ps_output  LeftPortType=input  RightPortType=output  PseudoPeriodic=off  Frequencies=[]  VectorFormat=1-D array  Unit=mm/s  AffineConversion=off
  PS-Simulink Converter8 : nesl_utility/PS-Simulink Converter  PhysicalDomain=network_engine_domain  SubClassName=ps_output  LeftPortType=input  RightPortType=output  PseudoPeriodic=off  Frequencies=[]  VectorFormat=1-D array  Unit=N  AffineConversion=off
  p : PMIOPort  Side=Left
  v : PMIOPort  Port=2  Side=Left
  f : PMIOPort  Port=3  Side=Left
  fc : PMIOPort  Port=4  Side=Left
  i : PMIOPort  Port=5  Side=Left
  m : Outport  VectorParamsAs1DForOutWhenUnconnected=off
  wires:
  Bus Creator/1 -> m/1  "b"
  PS-Simulink Converter8/1 -> Bus Creator/3  "f"
  PS-Simulink Converter7/1 -> Bus Creator/2  "v"
  PS-Simulink Converter/1 -> Bus Creator/1  "p"
  PS-Simulink Converter1/1 -> Bus Creator/4  "i"
  PS-Simulink Converter2/1 -> Bus Creator/5  "fc"
  connections:
  PS-Simulink Converter8/LConn1 -- f/RConn1
  PS-Simulink Converter7/LConn1 -- v/RConn1
  PS-Simulink Converter/LConn1 -- p/RConn1
  PS-Simulink Converter1/LConn1 -- i/RConn1
  PS-Simulink Converter2/LConn1 -- fc/RConn1

== system youBot_Arm_recovery/Arm/Actuation/Motor/Forearm/Ideal ==
  C : Inport
  Current Source : fl_lib/Electrical/Electrical Sources/Controlled Current Source
  Meas F : Subsystem
      mask Display: disp('m')
  PS Abs : MyMath_lib/PS Abs
      settings: InternalSimscapePortConfiguration="{\"Bottom\":[],\"Left\":[{\"id\":\"I\",\"label\":\"\",\"type\":\"input\"}],\"Right\":[{\"id\":\"O\",\"label\":\"\",\"type\":\"output\"}],\"Top\":[]}"
  PS Motor Const : fl_lib/Physical Signals/Functions/PS Gain  gain=YBT_Par.Forearm.Motor.K/YBT_Par.Forearm.Motor.gr s^2 / (kg*m^2)
  Resistor : fl_lib/Electrical/Electrical Elements/Resistor  R=YBT_Par.Forearm.Motor.R Ohm  i_specify=off  i_priority=None  i=0 A  i_nominal_specify=off  i_nominal_value=1  i_nominal_unit=A  v_specify=off  v_priority=None  v=0 V  v_nominal_specify=off  v_nominal_value=1  v_nominal_unit=V
  RevoluteBicepForearm : sm_lib/Joints/Revolute Joint  JointMode=Normal  CompositeWrenchDir=FollowerOnBase  CompositeWrenchFrame=BaseFrame  SenseConstraintForce=on  SenseConstraintTorque=off  SenseTotalForce=off  SenseTotalTorque=off  PositionTargetSpecify=on  PositionTargetPriority=Low  PositionTargetValue=smiData.RevoluteJoint(2).Rz.Pos  PositionTargetValueUnits=deg  VelocityTargetSpecify=off  VelocityTargetPriority=High  VelocityTargetValue=0  VelocityTargetValueUnits=deg/s  EquilibriumPosition=0  EquilibriumPositionUnits=rad  SpringStiffness=0  SpringStiffnessUnits=N*m/rad  DampingCoefficient=YBT_Par.Forearm.Motor.friction  DampingCoefficientUnits=N*m/(rad/s)  LowerLimitSpecify=off  LowerLimitBound=-90  LowerLimitBoundUnits=deg  LowerLimitStiffness=1e4  LowerLimitStiffnessUnits=N*m/deg  LowerLimitDamping=10  LowerLimitDampingUnits=N*m/(deg/s)  LowerLimitTransitionRegionWidth=0.1  LowerLimitTransitionRegionWidthUnits=deg  UpperLimitSpecify=off  UpperLimitBound=90  UpperLimitBoundUnits=deg  UpperLimitStiffness=1e4  UpperLimitStiffnessUnits=N*m/deg  UpperLimitDamping=10  UpperLimitDampingUnits=N*m/(deg/s)  UpperLimitTransitionRegionWidth=0.1  UpperLimitTransitionRegionWidthUnits=deg  TorqueActuationMode=ComputedTorque  MotionActuationMode=InputMotion  SensePosition=on  SenseVelocity=on  SenseAcceleration=off  SenseTorqueForce=on  SenseLowerLimitTorqueForce=off  SenseUpperLimitTorqueForce=off
  Simulink-PS Converter1 : nesl_utility/Simulink-PS Converter  Tag=CustomStyle  PhysicalDomain=network_engine_domain  SubClassName=ps_input  LeftPortType=input  RightPortType=output  PseudoPeriodic=off  Frequencies=[]  NoiseDistribution=none  NoiseParameters=[]  Unit=deg  AffineConversion=off  FilteringAndDerivatives=filter  SimscapeFilterOrder=2  InputFilterTimeConstant=0.005  UdotUserProvided=1
  B : PMIOPort  Side=Left
  F : PMIOPort  Port=2  Side=Right
  + : PMIOPort  Port=3  Side=Left
  - : PMIOPort  Port=4  Side=Right
  m : Outport  VectorParamsAs1DForOutWhenUnconnected=off
  wires:
  Meas F/1(F) -> m/1
  C/1 -> Simulink-PS Converter1/1
  connections:
  Resistor/LConn1 -- Current Source/LConn1
  PS Abs/RConn1 -- Meas F/LConn5 -- Current Source/RConn1
  PS Motor Const/RConn1 -- PS Abs/LConn1
  -/RConn1 -- Resistor/RConn1
  RevoluteBicepForearm/RConn3 -- Meas F/LConn2
  Meas F/LConn3 -- PS Motor Const/LConn1 -- RevoluteBicepForearm/RConn4
  RevoluteBicepForearm/RConn2 -- Meas F/LConn1
  Current Source/RConn2 -- +/RConn1
  RevoluteBicepForearm/LConn2 -- Simulink-PS Converter1/RConn1
  RevoluteBicepForearm/LConn1 -- B/RConn1
  RevoluteBicepForearm/RConn1 -- F/RConn1
  RevoluteBicepForearm/RConn5 -- Meas F/LConn4

== system youBot_Arm_recovery/Arm/Actuation/Motor/Forearm/Motor ==
  C : Inport
  Meas P : Subsystem  Tag=CustomStyle
      mask Display: disp('m')
  Motor : Motor_Lib/Motor  Tag=PublishSubsystem  VariantControl=Motor  r_motor=YBT_Par.Forearm.Motor.R  l_motor=YBT_Par.Forearm.Motor.L  k_motor=1/YBT_Par.Forearm.Motor.K  i_motor_noLoad=YBT_Par.Forearm.Motor.no_load_i  v_supply=YBT_Par.Battery.v  gear_ratio=YBT_Par.Forearm.Motor.gr  friction_visc=YBT_Par.Forearm.Motor.friction  ctrl_deadZone=YBT_Par.Control.Dead_Band
  RevoluteBicepForearm : sm_lib/Joints/Revolute Joint  JointMode=Normal  CompositeWrenchDir=FollowerOnBase  CompositeWrenchFrame=BaseFrame  SenseConstraintForce=on  SenseConstraintTorque=off  SenseTotalForce=off  SenseTotalTorque=off  PositionTargetSpecify=on  PositionTargetPriority=Low  PositionTargetValue=smiData.RevoluteJoint(2).Rz.Pos  PositionTargetValueUnits=deg  VelocityTargetSpecify=off  VelocityTargetPriority=High  VelocityTargetValue=0  VelocityTargetValueUnits=deg/s  EquilibriumPosition=0  EquilibriumPositionUnits=rad  SpringStiffness=0  SpringStiffnessUnits=N*m/rad  DampingCoefficient=0  DampingCoefficientUnits=N*m/(rad/s)  LowerLimitSpecify=off  LowerLimitBound=-90  LowerLimitBoundUnits=deg  LowerLimitStiffness=1e4  LowerLimitStiffnessUnits=N*m/deg  LowerLimitDamping=10  LowerLimitDampingUnits=N*m/(deg/s)  LowerLimitTransitionRegionWidth=0.1  LowerLimitTransitionRegionWidthUnits=deg  UpperLimitSpecify=off  UpperLimitBound=90  UpperLimitBoundUnits=deg  UpperLimitStiffness=1e4  UpperLimitStiffnessUnits=N*m/deg  UpperLimitDamping=10  UpperLimitDampingUnits=N*m/(deg/s)  UpperLimitTransitionRegionWidth=0.1  UpperLimitTransitionRegionWidthUnits=deg  TorqueActuationMode=InputTorque  MotionActuationMode=ComputedMotion  SensePosition=on  SenseVelocity=on  SenseAcceleration=off  SenseTorqueForce=on  SenseLowerLimitTorqueForce=off  SenseUpperLimitTorqueForce=off
  Sensing i : Subsystem
      mask Display: disp('i')
  B : PMIOPort  Side=Left
  F : PMIOPort  Port=2  Side=Right
  - : PMIOPort  Port=3  Side=Right
  + : PMIOPort  Port=4  Side=Left
  m : Outport  VectorParamsAs1DForOutWhenUnconnected=off
  wires:
  Meas P/1(m) -> m/1
  C/1 -> Motor/1
  connections:
  RevoluteBicepForearm/RConn2 -- Motor/RConn1 -- Meas P/LConn1
  RevoluteBicepForearm/RConn4 -- Meas P/LConn3
  RevoluteBicepForearm/RConn3 -- Motor/RConn2 -- Meas P/LConn2
  RevoluteBicepForearm/LConn2 -- Motor/LConn1
  RevoluteBicepForearm/RConn1 -- F/RConn1
  RevoluteBicepForearm/LConn1 -- B/RConn1
  Motor/RConn3 -- Sensing i/LConn1
  Motor/LConn2 -- +/RConn1
  Sensing i/RConn2 -- -/RConn1
  Sensing i/RConn1 -- Meas P/LConn5
  RevoluteBicepForearm/RConn5 -- Meas P/LConn4

== system youBot_Arm_recovery/Arm/Actuation/Motor/Gripper/Ideal ==
  C : Inport
  Current Source : fl_lib/Electrical/Electrical Sources/Controlled Current Source
  Meas G : Subsystem
      mask Display: disp('m')
  PS Abs : MyMath_lib/PS Abs
      settings: InternalSimscapePortConfiguration="{\"Bottom\":[],\"Left\":[{\"id\":\"I\",\"label\":\"\",\"type\":\"input\"}],\"Right\":[{\"id\":\"O\",\"label\":\"\",\"type\":\"output\"}],\"Top\":[]}"
  PS Motor Const : fl_lib/Physical Signals/Functions/PS Gain  gain=YBT_Par.Gripper.Motor.K/YBT_Par.Gripper.Motor.gr s^2 / (kg*m^2)
  Resistor : fl_lib/Electrical/Electrical Elements/Resistor  R=YBT_Par.Gripper.Motor.R Ohm  i_specify=off  i_priority=None  i=0 A  i_nominal_specify=off  i_nominal_value=1  i_nominal_unit=A  v_specify=off  v_priority=None  v=0 V  v_nominal_specify=off  v_nominal_value=1  v_nominal_unit=V
  RevoluteWristGripperPivot : sm_lib/Joints/Revolute Joint  JointMode=Normal  CompositeWrenchDir=FollowerOnBase  CompositeWrenchFrame=BaseFrame  SenseConstraintForce=on  SenseConstraintTorque=off  SenseTotalForce=off  SenseTotalTorque=off  PositionTargetSpecify=on  PositionTargetPriority=Low  PositionTargetValue=smiData.RevoluteJoint(4).Rz.Pos  PositionTargetValueUnits=deg  VelocityTargetSpecify=off  VelocityTargetPriority=High  VelocityTargetValue=0  VelocityTargetValueUnits=deg/s  EquilibriumPosition=0  EquilibriumPositionUnits=rad  SpringStiffness=0  SpringStiffnessUnits=N*m/rad  DampingCoefficient=YBT_Par.Gripper.Motor.friction  DampingCoefficientUnits=N*m/(rad/s)  LowerLimitSpecify=off  LowerLimitBound=-90  LowerLimitBoundUnits=deg  LowerLimitStiffness=1e4  LowerLimitStiffnessUnits=N*m/deg  LowerLimitDamping=10  LowerLimitDampingUnits=N*m/(deg/s)  LowerLimitTransitionRegionWidth=0.1  LowerLimitTransitionRegionWidthUnits=deg  UpperLimitSpecify=off  UpperLimitBound=90  UpperLimitBoundUnits=deg  UpperLimitStiffness=1e4  UpperLimitStiffnessUnits=N*m/deg  UpperLimitDamping=10  UpperLimitDampingUnits=N*m/(deg/s)  UpperLimitTransitionRegionWidth=0.1  UpperLimitTransitionRegionWidthUnits=deg  TorqueActuationMode=ComputedTorque  MotionActuationMode=InputMotion  SensePosition=on  SenseVelocity=on  SenseAcceleration=off  SenseTorqueForce=on  SenseLowerLimitTorqueForce=off  SenseUpperLimitTorqueForce=off
  Simulink-PS Converter2 : nesl_utility/Simulink-PS Converter  Tag=CustomStyle  PhysicalDomain=network_engine_domain  SubClassName=ps_input  LeftPortType=input  RightPortType=output  PseudoPeriodic=off  Frequencies=[]  NoiseDistribution=none  NoiseParameters=[]  Unit=deg  AffineConversion=off  FilteringAndDerivatives=filter  SimscapeFilterOrder=2  InputFilterTimeConstant=0.005  UdotUserProvided=1
  B : PMIOPort  Side=Left
  F : PMIOPort  Port=2  Side=Right
  + : PMIOPort  Port=3  Side=Left
  - : PMIOPort  Port=4  Side=Right
  m : Outport  VectorParamsAs1DForOutWhenUnconnected=off
  wires:
  Meas G/1(G) -> m/1
  C/1 -> Simulink-PS Converter2/1
  connections:
  PS Motor Const/RConn1 -- PS Abs/LConn1
  Resistor/LConn1 -- Current Source/LConn1
  PS Abs/RConn1 -- Meas G/LConn5 -- Current Source/RConn1
  +/RConn1 -- Current Source/RConn2
  RevoluteWristGripperPivot/RConn2 -- Meas G/LConn1
  RevoluteWristGripperPivot/RConn3 -- Meas G/LConn2
  RevoluteWristGripperPivot/LConn2 -- Simulink-PS Converter2/RConn1
  Meas G/LConn3 -- PS Motor Const/LConn1 -- RevoluteWristGripperPivot/RConn4
  RevoluteWristGripperPivot/LConn1 -- B/RConn1
  RevoluteWristGripperPivot/RConn1 -- F/RConn1
  Resistor/RConn1 -- -/RConn1
  RevoluteWristGripperPivot/RConn5 -- Meas G/LConn4

== system youBot_Arm_recovery/Arm/Actuation/Motor/Gripper/Motor ==
  C : Inport
  Meas P : Subsystem  Tag=CustomStyle
      mask Display: disp('m')
  Motor : Motor_Lib/Motor  VariantControl=Motor  r_motor=YBT_Par.Gripper.Motor.R  l_motor=YBT_Par.Gripper.Motor.L  k_motor=1/YBT_Par.Gripper.Motor.K  i_motor_noLoad=YBT_Par.Gripper.Motor.no_load_i  v_supply=YBT_Par.Battery.v  gear_ratio=YBT_Par.Gripper.Motor.gr  friction_visc=YBT_Par.Gripper.Motor.friction  ctrl_deadZone=YBT_Par.Control.Dead_Band
  RevoluteWristGripperPivot : sm_lib/Joints/Revolute Joint  JointMode=Normal  CompositeWrenchDir=FollowerOnBase  CompositeWrenchFrame=BaseFrame  SenseConstraintForce=on  SenseConstraintTorque=off  SenseTotalForce=off  SenseTotalTorque=off  PositionTargetSpecify=on  PositionTargetPriority=Low  PositionTargetValue=smiData.RevoluteJoint(4).Rz.Pos  PositionTargetValueUnits=deg  VelocityTargetSpecify=off  VelocityTargetPriority=High  VelocityTargetValue=0  VelocityTargetValueUnits=deg/s  EquilibriumPosition=0  EquilibriumPositionUnits=rad  SpringStiffness=0  SpringStiffnessUnits=N*m/rad  DampingCoefficient=0  DampingCoefficientUnits=N*m/(rad/s)  LowerLimitSpecify=off  LowerLimitBound=-90  LowerLimitBoundUnits=deg  LowerLimitStiffness=1e4  LowerLimitStiffnessUnits=N*m/deg  LowerLimitDamping=10  LowerLimitDampingUnits=N*m/(deg/s)  LowerLimitTransitionRegionWidth=0.1  LowerLimitTransitionRegionWidthUnits=deg  UpperLimitSpecify=off  UpperLimitBound=90  UpperLimitBoundUnits=deg  UpperLimitStiffness=1e4  UpperLimitStiffnessUnits=N*m/deg  UpperLimitDamping=10  UpperLimitDampingUnits=N*m/(deg/s)  UpperLimitTransitionRegionWidth=0.1  UpperLimitTransitionRegionWidthUnits=deg  TorqueActuationMode=InputTorque  MotionActuationMode=ComputedMotion  SensePosition=on  SenseVelocity=on  SenseAcceleration=off  SenseTorqueForce=on  SenseLowerLimitTorqueForce=off  SenseUpperLimitTorqueForce=off
  Sensing i : Subsystem
      mask Display: disp('i')
  B : PMIOPort  Side=Left
  F : PMIOPort  Port=2  Side=Right
  - : PMIOPort  Port=3  Side=Right
  + : PMIOPort  Port=4  Side=Left
  m : Outport  VectorParamsAs1DForOutWhenUnconnected=off
  wires:
  Meas P/1(m) -> m/1
  C/1 -> Motor/1
  connections:
  RevoluteWristGripperPivot/RConn2 -- Motor/RConn1 -- Meas P/LConn1
  RevoluteWristGripperPivot/RConn4 -- Meas P/LConn3
  RevoluteWristGripperPivot/RConn3 -- Motor/RConn2 -- Meas P/LConn2
  RevoluteWristGripperPivot/LConn2 -- Motor/LConn1
  RevoluteWristGripperPivot/RConn1 -- F/RConn1
  RevoluteWristGripperPivot/LConn1 -- B/RConn1
  Sensing i/LConn1 -- Motor/RConn3
  Motor/LConn2 -- +/RConn1
  Sensing i/RConn2 -- -/RConn1
  Meas P/LConn5 -- Sensing i/RConn1
  RevoluteWristGripperPivot/RConn5 -- Meas P/LConn4
